simulink model "Practical2_Quadrotor"  (R2026b)
settings: Solver=ode45  StopTime=2  MaxStep=0.01  RelTol=1e-6  AbsTol=1e-8
values from neighbouring files (symbols this model uses):
  c_drag = 0    [practical2_parameters.m]    (also in run_section7_tests.m)
  g = 9.81    [practical2_parameters.m]
  J = diag(Jdiag)    [practical2_parameters.m]
  kM = kMT*kT    [practical2_parameters.m]
  kT = 2*m_nom*g/(4*Omega_max^2)    [practical2_parameters.m]
  m = m_nom    [practical2_parameters.m]    (also in run_section7_tests.m = 1.80*m0)
  Omega_cmd = Omega_hover*ones(4,1)    [practical2_parameters.m]    (also in run_section7_tests.m = sqrt(T_target/kT); run_validation_tests.m = sqrt(T_target/kT))
  Omega_max = 800    [practical2_parameters.m]
  rotor_xy = [d d -d -d; -d d d -d]    [practical2_parameters.m]
  sigma = [1;-1;1;-1]    [practical2_parameters.m]    (also in run_validation_tests.m = [1;-1;1;-1] produces +Mz and +r/+psi yaw acceleration with M)
  X0 = zeros(12,1)    [practical2_parameters.m]    (also in run_validation_tests.m)
settings Model: Creator=nicholas  LastModifiedBy=Nicholas Khor

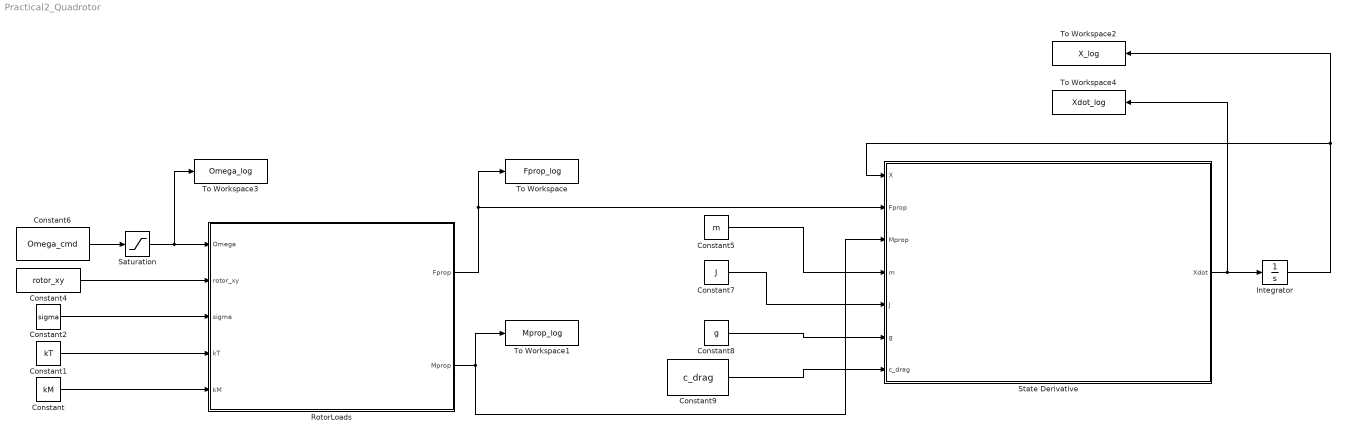
== system Practical2_Quadrotor ==
  Constant : Constant  Value=kM
  Constant1 : Constant  Value=kT
  Constant2 : Constant  Value=sigma
  Constant4 : Constant  Value=rotor_xy
  Constant5 : Constant  Value=m
  Constant6 : Constant  Value=Omega_cmd
  Constant7 : Constant  Value=J
  Constant8 : Constant  Value=g
  Constant9 : Constant  Value=c_drag
  Integrator : Integrator  InitialCondition=X0
  RotorLoads : MATLAB Function  TreatAsAtomicUnit=on
  Saturation : Saturate  UpperLimit=Omega_max  LowerLimit=0
  State Derivative : MATLAB Function  TreatAsAtomicUnit=on
  To Workspace : ToWorkspace  VariableName=Fprop_log  SaveFormat=Timeseries  SampleTime=0.01
  To Workspace1 : ToWorkspace  VariableName=Mprop_log  SaveFormat=Timeseries  SampleTime=0.01
  To Workspace2 : ToWorkspace  VariableName=X_log  SaveFormat=Timeseries  SampleTime=0.01
  To Workspace3 : ToWorkspace  VariableName=Omega_log  SaveFormat=Timeseries  SampleTime=0.01
  To Workspace4 : ToWorkspace  VariableName=Xdot_log  SaveFormat=Timeseries  SampleTime=0.01
  wires:
  Constant4/1 -> RotorLoads/2(rotor_xy)
  Constant2/1 -> RotorLoads/3(sigma)
  Saturation/1 -> To Workspace3/1, RotorLoads/1(Omega)
  Constant1/1 -> RotorLoads/4(kT)
  Constant/1 -> RotorLoads/5(kM)
  RotorLoads/1(Fprop) -> State Derivative/2(Fprop), To Workspace/1
  RotorLoads/2(Mprop) -> To Workspace1/1, State Derivative/3(Mprop)
  Constant5/1 -> State Derivative/4(m)
  Constant7/1 -> State Derivative/5(J)
  Constant8/1 -> State Derivative/6(g)
  Constant9/1 -> State Derivative/7(c_drag)
  State Derivative/1(Xdot) -> To Workspace4/1, Integrator/1
  Integrator/1 -> To Workspace2/1, State Derivative/1(X)
  Constant6/1 -> Saturation/1

== matlab function Practical2_Quadrotor/State Derivative ==
  data: X input; Xdot output; Fprop input; Mprop input; m input; J input; g input; c_drag input
function Xdot = StateDerivative(X,Fprop,Mprop,m,J,g,c_drag)
% Compute 12-state rigid-body quadrotor derivatives in NED / body axes.

% Extract states
vb    = X(4:6);
phi   = X(7);
theta = X(8);
psi   = X(9);
omega = X(10:12);

% Body-to-NED rotation matrix R = Rz * Ry * Rx
Rx = [1 0 0; 0 cos(phi) -sin(phi); 0 sin(phi) cos(phi)];
Ry = [cos(theta) 0 sin(theta); 0 1 0; -sin(theta) 0 cos(theta)];
Rz = [cos(psi) -sin(psi) 0; sin(psi) cos(psi) 0; 0 0 1];
R  = Rz * Ry * Rx;

% Position kinematics (NED)
pos_dot = R * vb;

% Translational dynamics (body axes)
Fg     = R.' * [0; 0; m*g];
Fdrag  = -c_drag * vb;
vb_dot = (Fg + Fprop + Fdrag)/m - cross(omega, vb);

% Attitude kinematics (Euler angle rates)
E = [1  sin(phi)*tan(theta)   cos(phi)*tan(theta);
    0  cos(phi)             -sin(phi);
    0  sin(phi)/cos(theta)   cos(phi)/cos(theta)];
euler_dot = E * omega;

% Rotational dynamics (body axes)
omega_dot = J \ (Mprop - cross(omega, J * omega));

% Assemble 12x1 state derivative
Xdot = zeros(12,1);
Xdot(1:3)   = pos_dot;
Xdot(4:6)   = vb_dot;
Xdot(7:9)   = euler_dot;
Xdot(10:12) = omega_dot;
end

== matlab function Practical2_Quadrotor/RotorLoads ==
  data: Omega input; Fprop output; rotor_xy input; sigma input; kT input; kM input; Mprop output
function [Fprop,Mprop] = RotorLoads(Omega,rotor_xy,sigma,kT,kM)
% Sum the thrust forces and moments from all 4 rotors in body axes
% (x forward, y right, z down).

Fprop = zeros(3,1);
Mprop = zeros(3,1);

for i = 1:4
    Ti = kT * Omega(i)^2;
    Fi = [0; 0; -Ti];
    ri = [rotor_xy(1,i); rotor_xy(2,i); 0];
    Mi = cross(ri, Fi) + [0; 0; sigma(i) * kM * Omega(i)^2];

    Fprop = Fprop + Fi;
    Mprop = Mprop + Mi;
end
end
